simulink model "UkfObserverTest"  (R2026b)
settings: Solver=FixedStepDiscrete  StopTime=ukfTestCfg.Duration  FixedStep=ukfCfg.Model.Ts
PostLoadFcn:
  | addpath(fullfile(fileparts(get_param(bdroot,'FileName')),'..','build_process'));initialize_ukf_test(bdroot);
model workspace (MAT data in the model file):
  fixtureTruth.time = [0 5e-05 0.0001 0.00015 0.0002 0.00025 0.0003 0.00035 0.0004 0.00045 0.0005 0.00055 ... (10001 elements, 10001x1)]
  fixtureTruth.theta = [0.7 0.73 0.76 0.79 0.82 0.85 0.88 0.91 0.94 0.97 1 1.03 ... (10001 elements, 10001x1)]
  fixtureTruth.omega = [600 600 600 600 600 600 600 600 600 600 600 600 ... (10001 elements, 10001x1)]
  fixtureTruth.current = [-1.28843537448 -1.33373927001 -1.37784289022 -1.42070654484 -1.46229165945 -1.50256081028 -1.5414777578 -1.57900747938 -1.61511620081 -1.64977142668 -1.68294196962 -1.71459797838 ... (20002 elements, 10001x2)]
  fixtureTruth.voltage = [-15.090599744 -15.5653412529 -16.0260750053 -16.472386372 -16.9038737027 -17.3201486881 -17.7208367088 -18.1055771726 -18.4740238389 -18.8258451308 -19.1607244328 -19.4783603761 ... (20002 elements, 10001x2)]
  fixtureTruth.id = [0 0 0 0 0 0 0 0 0 0 0 0 ... (10001 elements, 10001x1)]
  fixtureTruth.iq = [2 2 2 2 2 2 2 2 2 2 2 2 ... (10001 elements, 10001x1)]
  fixtureTruth.motor.Ts = 5e-05
  fixtureTruth.motor.Rs = 0.5
  fixtureTruth.motor.L = 0.001
  fixtureTruth.motor.Flux = 0.035
  fixtureTruth.motor.PolePairs = 4
  fixtureTruth.direction_prior = [1 1 1 1 1 1 1 1 1 1 1 1 ... (10001 elements, 10001x1)]
  testStim.time = [0 5e-05 0.0001 0.00015 0.0002 0.00025 0.0003 0.00035 0.0004 0.00045 0.0005 0.00055 ... (10001 elements, 10001x1)]
  testStim.signals.values = [-15.090599744 -15.5653412529 -16.0260750053 -16.472386372 -16.9038737027 -17.3201486881 -17.7208367088 -18.1055771726 -18.4740238389 -18.8258451308 -19.1607244328 -19.4783603761 ... (90009 elements, 10001x9)]
  testStim.signals.dimensions = 9
  ukfCfg.Model.Ts = 5e-05
  ukfCfg.Model.Rs = 0.5
  ukfCfg.Model.L = 0.001
  ukfCfg.Model.Flux = 0.035
  ukfCfg.Model.PolePairs = 4
  ukfCfg.InitialOmega = 300
  ukfCfg.InitialAngle = 0
  ukfCfg.InitialStd = [1; 1; 500; 0.5]
  ukfCfg.ProcessNoiseDensity = [2; 2; 2000; 1e-05]
  ukfCfg.MeasurementStd = [0.002; 0.002]
  ukfCfg.QualificationTime = 0.02
  ukfCfg.MinOmega = 30
  ukfCfg.MinEmf = 1
  ukfCfg.MaxNIS = 25
  ukfCfg.MaxThetaStd = 0.12
  ukfCfg.MaxOmegaStd = 100
  ukfCfg.AngleRateTimeConstant = 0.002
  ukfCfg.MaxRateMismatch = 60
  ukfCfg.MaxOmega = 2000
  ukfCfg.MaxInputCurrent = 100
  ukfCfg.MaxInputVoltage = 1000
  ukfCfg.InitialVariance = [1; 1; 250000; 0.25]
  ukfCfg.ProcessVariance = [0.0001; 0.0001; 0.1; 5e-10]
  ukfCfg.MeasurementVariance = [4e-06; 4e-06]
  ukfCfg.QualificationSamples = 400
  ukfCfg.AngleRateAlpha = 0.0243902439024
  ukfCfg.Settings = [5e-05; 0.5; 0.001; 0.035; 300; 0; 1; 1; 250000; 0.25; 0.0001; 0.0001; 0.1; 5e-10; 4e-06; 4e-06; 400; 30; 1; 25; 0.12; 100; 0.0243902439024; 60; 2000; 100; 1000]
  ukfCfg.Alpha = 1
  ukfCfg.Beta = 2
  ukfCfg.Kappa = 0
  ukfCfg.StateScales = [1; 1; 100; 1]
  ukfCfg.InitialJitter = 1e-12
  ukfCfg.MaximumJitter = 1e-08
  ukfCfg.MaximumJitterAttempts = 5
  ukfCfg.MinimumAngleResultant = 1e-06
  ukfCfg.MaximumSigmaAngleDeviation = 1.56979632679
  ukfCfg.UnscentedSettings = [5e-05; 0.5; 0.001; 0.035; 300; 0; 1; 1; 250000; 0.25; 0.0001; 0.0001; 0.1; 5e-10; 4e-06; 4e-06; 400; 30; 1; 25; 0.12; 100; 0.0243902439024; 60; 2000; 100; 1000; 1; 2; 0; 1; 1; 100; 1; 1e-12; 1e-08; 5; 1e-06; 1.56979632679]
  ukfCfg.SigmaScale = 4
  ukfCfg.MeanWeights = [0; 0.125; 0.125; 0.125; 0.125; 0.125; 0.125; 0.125; 0.125]
  ukfCfg.CovarianceWeights = [2; 0.125; 0.125; 0.125; 0.125; 0.125; 0.125; 0.125; 0.125]
  ukfTestCfg.Duration = 0.5
  ukfTestCfg.InitialAngle = 0.7
  ukfTestCfg.ElectricalSpeed = 600
  ukfTestCfg.Id = 0
  ukfTestCfg.Iq = 2
  ukfTestCfg.Direction = 1
  ukfTestCfg.Enable = 1
  ukfTestCfg.Reset = 0
  ukfTestCfg.NoiseRms = 0
  ukfTestCfg.NoiseSeed = 42
  ukfTestCfg.CurrentDelay = 0
  ukfTestCfg.CheckStart = 0.35
  ukfTestCfg.AngleRmsLimit = 0.08
  ukfTestCfg.SpeedRmsLimit = 8
  ukfTestCfg.ValidFractionMinimum = 0.95
libraries: UkfObserver x1
settings Model: Creator=24322  LastModifiedBy=24322

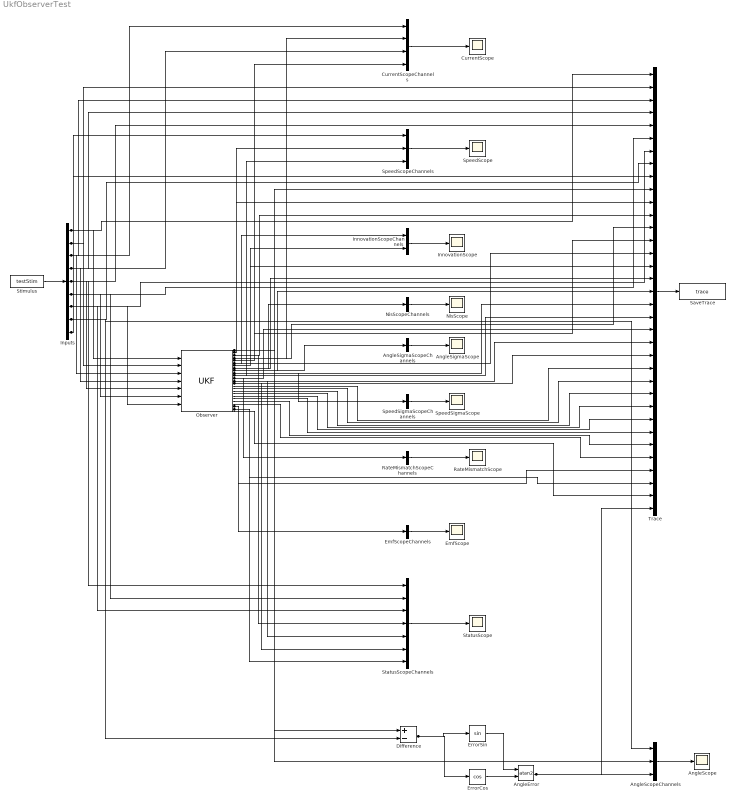
== system UkfObserverTest ==
  AngleError : Trigonometry  Operator=atan2
  AngleScope : Scope
  AngleScopeChannels : Mux  Inputs=3
  AngleSigmaScope : Scope
  AngleSigmaScopeChannels : Mux  Inputs=1
  CurrentScope : Scope
  CurrentScopeChannels : Mux
  Difference : Sum  Inputs=+-
  EmfScope : Scope
  EmfScopeChannels : Mux  Inputs=1
  ErrorCos : Trigonometry  Operator=cos
  ErrorSin : Trigonometry
  InnovationScope : Scope
  InnovationScopeChannels : Mux  Inputs=2
  Inputs : Demux  Outputs=9
  NisScope : Scope
  NisScopeChannels : Mux  Inputs=1
  Observer : UkfObserver/UKF  cfg=ukfCfg
  RateMismatchScope : Scope
  RateMismatchScopeChannels : Mux  Inputs=1
  SaveTrace : ToWorkspace  VariableName=trace  SaveFormat=Structure With Time  SampleTime=ukfCfg.Model.Ts
  SpeedScope : Scope
  SpeedScopeChannels : Mux  Inputs=3
  SpeedSigmaScope : Scope
  SpeedSigmaScopeChannels : Mux  Inputs=1
  StatusScope : Scope
  StatusScopeChannels : Mux  Inputs=7
  Stimulus : FromWorkspace  VariableName=testStim  SampleTime=ukfCfg.Model.Ts  Interpolate=off  OutputAfterFinalValue=Holding final value
  Trace : Mux  Inputs=35
  wires:
  StatusScopeChannels/1 -> StatusScope/1
  EmfScopeChannels/1 -> EmfScope/1
  RateMismatchScopeChannels/1 -> RateMismatchScope/1
  SpeedSigmaScopeChannels/1 -> SpeedSigmaScope/1
  AngleSigmaScopeChannels/1 -> AngleSigmaScope/1
  NisScopeChannels/1 -> NisScope/1
  InnovationScopeChannels/1 -> InnovationScope/1
  CurrentScopeChannels/1 -> CurrentScope/1
  SpeedScopeChannels/1 -> SpeedScope/1
  AngleScopeChannels/1 -> AngleScope/1
  Observer/24 -> Trace/33, StatusScopeChannels/7
  Observer/23 -> Trace/32, EmfScopeChannels/1
  Observer/22 -> Trace/31
  Observer/21 -> Trace/30
  Observer/20 -> Trace/29
  Observer/19 -> Trace/28
  Observer/18 -> Trace/27
  Observer/17 -> Trace/26
  Observer/16 -> Trace/25
  Observer/15 -> Trace/24
  Observer/14 -> Trace/23, StatusScopeChannels/6
  Observer/13 -> Trace/22, StatusScopeChannels/5
  Observer/12 -> Trace/21, RateMismatchScopeChannels/1
  Observer/11 -> Trace/20, SpeedScopeChannels/3
  Observer/10 -> Trace/19, SpeedSigmaScopeChannels/1
  Observer/9 -> Trace/18, AngleSigmaScopeChannels/1
  Observer/8 -> Trace/17, NisScopeChannels/1
  Observer/7 -> Trace/16, InnovationScopeChannels/2
  Observer/6 -> Trace/15, InnovationScopeChannels/1
  Observer/5 -> Trace/14, CurrentScopeChannels/4
  Observer/4 -> Trace/13, CurrentScopeChannels/2
  Observer/3 -> Trace/12, StatusScopeChannels/4
  Observer/2 -> Trace/11, SpeedScopeChannels/2
  Inputs/9 -> Trace/9, SpeedScopeChannels/1
  Inputs/7 -> Observer/7, Trace/7, StatusScopeChannels/3
  Inputs/6 -> Observer/6, Trace/6, StatusScopeChannels/2
  Inputs/5 -> Trace/5, Observer/5, StatusScopeChannels/1
  Inputs/4 -> Trace/4, Observer/4, CurrentScopeChannels/3
  Inputs/3 -> Trace/3, Observer/3, CurrentScopeChannels/1
  Inputs/2 -> Observer/2, Trace/2
  Inputs/1 -> Observer/1, Trace/1
  Trace/1 -> SaveTrace/1
  Observer/25 -> Trace/34
  AngleError/1 -> Trace/35, AngleScopeChannels/3
  ErrorCos/1 -> AngleError/2
  ErrorSin/1 -> AngleError/1
  Difference/1 -> ErrorSin/1, ErrorCos/1
  Inputs/8 -> Trace/8, Difference/2, AngleScopeChannels/1
  Observer/1 -> Difference/1, Trace/10, AngleScopeChannels/2
  Stimulus/1 -> Inputs/1
